simulink model "Lab2_Task_2"  (R2025b)
settings: Solver=FixedStepAuto  StartTime=0.0  StopTime=inf  RelTol=1e-3
model workspace (MAT data in the model file):
  SL_ROS_VariableLengthArrays_MaxSizes.CommonInfo.ArrayTruncateAction = 'EmitWarning'
  SL_ROS_VariableLengthArrays_MaxSizes.MsgTypeMap = containers.Map
  SL_ROS_VariableLengthArrays_MaxSizes.MsgTypeMap.serialization.keys = {'sensor_msgs/LaserScan'}
  SL_ROS_VariableLengthArrays_MaxSizes.MsgTypeMap.serialization.values{1}(1).PropertyName = 'intensities'
  SL_ROS_VariableLengthArrays_MaxSizes.MsgTypeMap.serialization.values{1}(1).DataType = 'single'
  SL_ROS_VariableLengthArrays_MaxSizes.MsgTypeMap.serialization.values{1}(1).MaxLength = 360
  SL_ROS_VariableLengthArrays_MaxSizes.MsgTypeMap.serialization.values{1}(2).PropertyName = 'ranges'
  SL_ROS_VariableLengthArrays_MaxSizes.MsgTypeMap.serialization.values{1}(2).DataType = 'single'
  SL_ROS_VariableLengthArrays_MaxSizes.MsgTypeMap.serialization.values{1}(2).MaxLength = 360
  SL_ROS_VariableLengthArrays_MaxSizes.MsgTypeMap.serialization.uniformity = 0
  SL_ROS_VariableLengthArrays_MaxSizes.MsgTypeMap.serialization.keyType = 'char'
  SL_ROS_VariableLengthArrays_MaxSizes.MsgTypeMap.serialization.valueType = 'any'
undefined symbols (not defined in the file or in its folder): header, twist
libraries: ros2lib x4
settings Model: Creator=scott  LastModifiedBy=abodynasser22
settings OptimizationCC: DefaultParameterBehavior=Inlined  EnhancedBackFolding=on  PassReuseOutputArgsAs=Individual arguments  ZeroExternalMemoryAtStartup=off  ZeroInternalMemoryAtStartup=off  MaxStackSize=64  OptimizeBlockOrder=speed  DifferentSizesBufferReuse=on  OptimizationCustomize=off  EfficientTunableParamExpr=on
settings DebuggingCC: ParameterTunabilityLossMsg=error
settings HardwareCC: ProdBitPerPointer=32.0  ProdBitPerSizeT=32.0  ProdBitPerPtrDiffT=32.0  ProdWordSize=32.0  ProdHWDeviceType=Intel->x86-32 (Windows32)  UseEmbeddedCoderFeatures=off
settings SFSimCC: MATLABDynamicMemAlloc=off
settings RTWCC: SystemTargetFile=ert.tlc  HardwareBoard=Robot Operating System 2 (ROS 2)  TLCOptions="-aInlineSetEventsForThisBaseRateFcn=TLC_FALSE -aSuppressMultiTaskScheduler=TLC_FALSE  -aRateBasedStepFcn=0"  TemplateMakefile=ert_default_tmf  Toolchain=Colcon Tools  TargetLang=C++  Description=Embedded Coder
settings CodeAppCC: ForceParamTrailComments=on  IgnoreCustomStorageClasses=off  OperatorAnnotations=on  SimulinkDataObjDesc=on  SFDataObjDesc=on  InsertBlockDesc=on
settings ERTTargetCC: ExtModeTransport=2.0  ExtModeStaticAlloc=on  ExtModeAutomaticAllocSize=off  ExtModeMexFile=ext_xcp  ExtModeIntrfLevel=Level2 - Open  RootIOFormat=Structure reference  CodeInterfacePackaging=C++ class  SupportNonInlinedSFcns=on

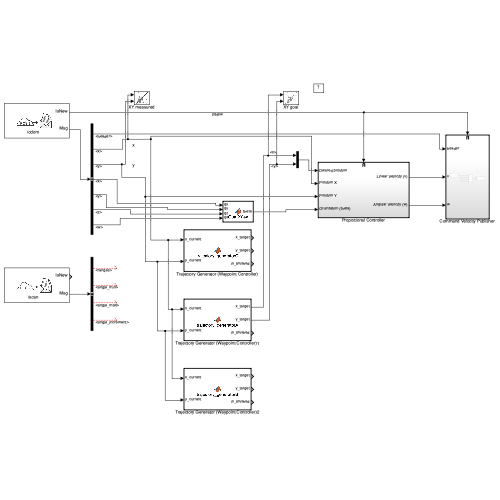
[thumbnail: Simulink's stored preview of the top-level diagram]
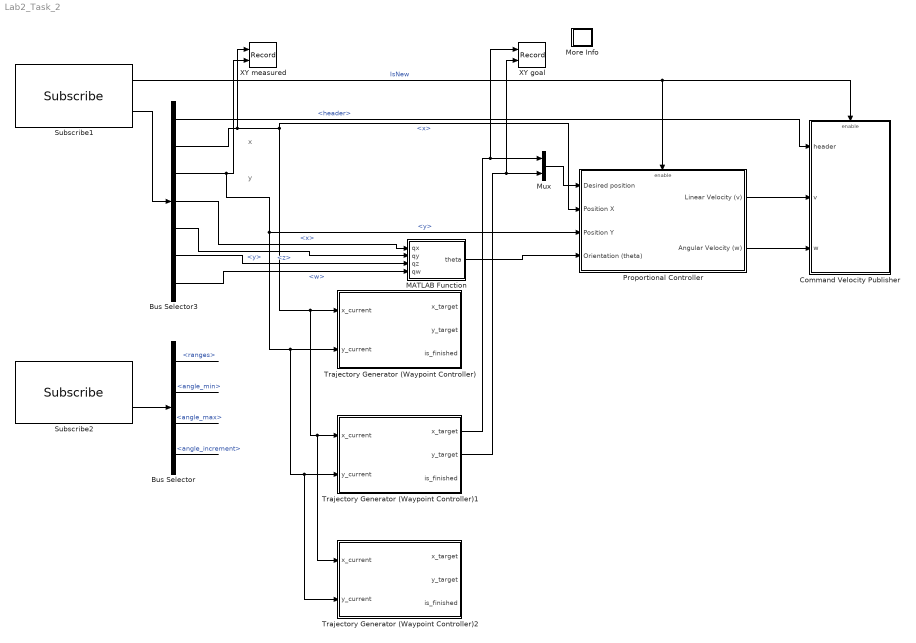
== system Lab2_Task_2 ==
  note: y
  note: x
  Bus Selector : BusSelector  OutputSignals=ranges,angle_min,angle_max,angle_increment
  Bus Selector3 : BusSelector  OutputSignals=header,pose.pose.position.x,pose.pose.position.y,pose.pose.orientation.x,pose.pose.orientation.y,pose.pose.orientation.z,pose.pose.orientation.w
  Command Velocity Publisher : Subsystem
  MATLAB Function : MATLAB Function  TreatAsAtomicUnit=on
  More Info : Subsystem
      settings: OpenFcn=showdemo(bdroot(gcb))
      mask Display: disp('?')
  Mux : Mux  Inputs=2
  Proportional Controller : Subsystem
  Subscribe1 : ros2lib/Subscribe  topicSource=Select from ROS network  topic=/odom  messageType=nav_msgs/Odometry  sampleTime=-1  QOSHistory=Keep last  QOSDepth=10  QOSReliability=Reliable  QOSDurability=Volatile  QOSDeadline=Inf  QOSLifespan=Inf  QOSLiveliness=Automatic  QOSLeaseDuration=Inf  QOSAvoidROSNamespaceConventions=off
  Subscribe2 : ros2lib/Subscribe  topicSource=Select from ROS network  topic=/scan  messageType=sensor_msgs/LaserScan  sampleTime=-1  QOSHistory=Keep last  QOSDepth=10  QOSReliability=Best effort  QOSDurability=Volatile  QOSDeadline=Inf  QOSLifespan=Inf  QOSLiveliness=Automatic  QOSLeaseDuration=Inf  QOSAvoidROSNamespaceConventions=off
  Trajectory Generator (Waypoint Controller) : MATLAB Function  TreatAsAtomicUnit=on
  Trajectory Generator (Waypoint Controller)1 : MATLAB Function  TreatAsAtomicUnit=on
  Trajectory Generator (Waypoint Controller)2 : MATLAB Function  TreatAsAtomicUnit=on
  XY goal : Record  NumPorts=2.0  FileSettingsInternal="{\"entries\":[{\"content\":{\"excelSettings\":{\"content\":{},\"type\":\"Streamout.ExcelSettings\"},\"parquetSettings\":{\"content\":{},\"type\":\"Streamout.ParquetSettings\"}},\"type\":\"Streamout.FileSettingStorage\",\"uuid\":\"\"}],\"packageUris\":[\"http:\\/\\/schema.mathworks.com\\/mf0\\/streamout_blocks\\/R2020a\"],\"version\":\"1.0\"}"  FrameSettings=[0, 0]  Layout=[1 1]  SignalsInternal="{\"entries\":[{\"content\":{\"signals\":[{\"content\":{\"blockPath\":[],\"dimensions\":[1],\"domain\":\"\",\"lineColor\":\"#a2142f\",\"plots\":[ 1 ],\"port\":1,\"signalID\":1,\"signalName\":\"<x>\"},\"type\":\"RecordBlkView.Signal\",\"uuid\":\"\"},{\"content\":{\"blockPath\":[],\"dimensions\":[1],\"domain\":\"\",\"lineColor\":\"#139fff\",\"plots\":[ 1 ],\"port\":2,\"signalID\":2,\"signalName\":\"<y>\"},\"type\":\"RecordBlkView.Signal\",\"uuid\":\"\"}]},\"type\":\"RecordBlkView.InputSignals\",\"uuid\":\"\"}],\"packageUris\":[\"http:\\/\\/schema.mathworks.com\\/mf0\\/streamout_blocks\\/R2020a\"],\"version\":\"1.0\"}"  VisualizationBindings="{\"xyplotplugin\":{\"info\":[{\"series\":[{\"bindingParametersList\":[{\"parameter\":\"X-Axis\",\"signalID\":1,\"signalName\":\"<x>;\"},{\"parameter\":\"Y-Axis\",\"signalID\":2,\"signalName\":\"<y>;\"}],\"seriesID\":0}],\"subplotID\":1}]}}"  CompatibilityTag=XY
  XY measured : Record  NumPorts=2.0  FileSettingsInternal="{\"entries\":[{\"content\":{\"excelSettings\":{\"content\":{},\"type\":\"Streamout.ExcelSettings\"},\"parquetSettings\":{\"content\":{},\"type\":\"Streamout.ParquetSettings\"}},\"type\":\"Streamout.FileSettingStorage\",\"uuid\":\"\"}],\"packageUris\":[\"http:\\/\\/schema.mathworks.com\\/mf0\\/streamout_blocks\\/R2020a\"],\"version\":\"1.0\"}"  FrameSettings=[0, 0]  Layout=[1 1]  SignalsInternal="{\"entries\":[{\"content\":{\"signals\":[{\"content\":{\"blockPath\":[],\"dimensions\":[1],\"domain\":\"\",\"lineColor\":\"#a2142f\",\"plots\":[ 1 ],\"port\":1,\"signalID\":1,\"signalName\":\"<x>\"},\"type\":\"RecordBlkView.Signal\",\"uuid\":\"\"},{\"content\":{\"blockPath\":[],\"dimensions\":[1],\"domain\":\"\",\"lineColor\":\"#139fff\",\"plots\":[ 1 ],\"port\":2,\"signalID\":2,\"signalName\":\"<y>\"},\"type\":\"RecordBlkView.Signal\",\"uuid\":\"\"}]},\"type\":\"RecordBlkView.InputSignals\",\"uuid\":\"\"}],\"packageUris\":[\"http:\\/\\/schema.mathworks.com\\/mf0\\/streamout_blocks\\/R2020a\"],\"version\":\"1.0\"}"  VisualizationBindings="{\"xyplotplugin\":{\"info\":[{\"series\":[{\"bindingParametersList\":[{\"parameter\":\"X-Axis\",\"signalID\":1,\"signalName\":\"<x>;\"},{\"parameter\":\"Y-Axis\",\"signalID\":2,\"signalName\":\"<y>;\"}],\"seriesID\":0}],\"subplotID\":1}]}}"  CompatibilityTag=XY
  wires:
  Subscribe1/2 -> Bus Selector3/1
  Subscribe1/1 -> Command Velocity Publisher/Enable, Proportional Controller/Enable  "IsNew"
  Proportional Controller/1(Linear Velocity (v)) -> Command Velocity Publisher/2(v)
  Proportional Controller/2(Angular Velocity (w)) -> Command Velocity Publisher/3(w)
  Bus Selector3/1 -> Command Velocity Publisher/1(header)  "<header>"
  Bus Selector3/2 -> XY measured/1, Trajectory Generator (Waypoint Controller)2/1(x_current), Trajectory Generator (Waypoint Controller)1/1(x_current), Trajectory Generator (Waypoint Controller)/1(x_current), Proportional Controller/2(Position X)  "<x>"
  Bus Selector3/3 -> XY measured/2, Trajectory Generator (Waypoint Controller)2/2(y_current), Trajectory Generator (Waypoint Controller)1/2(y_current), Trajectory Generator (Waypoint Controller)/2(y_current), Proportional Controller/3(Position Y)  "<y>"
  Bus Selector3/4 -> MATLAB Function/1(qx)  "<x>"
  Bus Selector3/5 -> MATLAB Function/2(qy)  "<y>"
  Bus Selector3/6 -> MATLAB Function/3(qz)  "<z>"
  Bus Selector3/7 -> MATLAB Function/4(qw)  "<w>"
  Subscribe2/2 -> Bus Selector/1
  Bus Selector/1 -> ?  "<ranges>"
  Bus Selector/2 -> ?  "<angle_min>"
  Bus Selector/3 -> ?  "<angle_max>"
  Bus Selector/4 -> ?  "<angle_increment>"
  MATLAB Function/1(theta) -> Proportional Controller/4(Orientation (theta))
  Mux/1 -> Proportional Controller/1(Desired position)
  Trajectory Generator (Waypoint Controller)1/1(x_target) -> XY goal/1, Mux/1
  Trajectory Generator (Waypoint Controller)1/2(y_target) -> XY goal/2, Mux/2

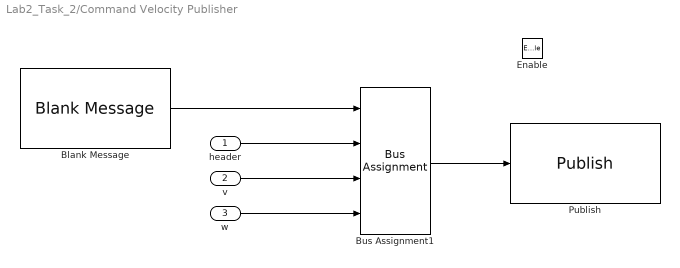
== system Lab2_Task_2/Command Velocity Publisher ==
  header : Inport
  v : Inport  Port=2
  w : Inport  Port=3
  Enable : EnablePort
  Blank Message : ros2lib/Blank Message  messageClass=Message  entityType=geometry_msgs/TwistStamped  messageType=geometry_msgs/TwistStamped  SampleTime=inf
  Bus Assignment1 : BusAssignment  DialogController=Simulink.DDGSource_BusAssignment  AssignedSignals=header,twist.linear.x,twist.angular.z
  Publish : ros2lib/Publish  topicSource=Select from ROS network  topic=/cmd_vel  messageType=geometry_msgs/TwistStamped  QOSHistory=Keep last  QOSDepth=10  QOSReliability=Reliable  QOSDurability=Volatile  QOSDeadline=Inf  QOSLifespan=Inf  QOSLiveliness=Automatic  QOSLeaseDuration=Inf  QOSAvoidROSNamespaceConventions=off
  wires:
  Bus Assignment1/1 -> Publish/1
  Blank Message/1 -> Bus Assignment1/1
  header/1 -> Bus Assignment1/2
  v/1 -> Bus Assignment1/3
  w/1 -> Bus Assignment1/4

== system Lab2_Task_2/More Info ==

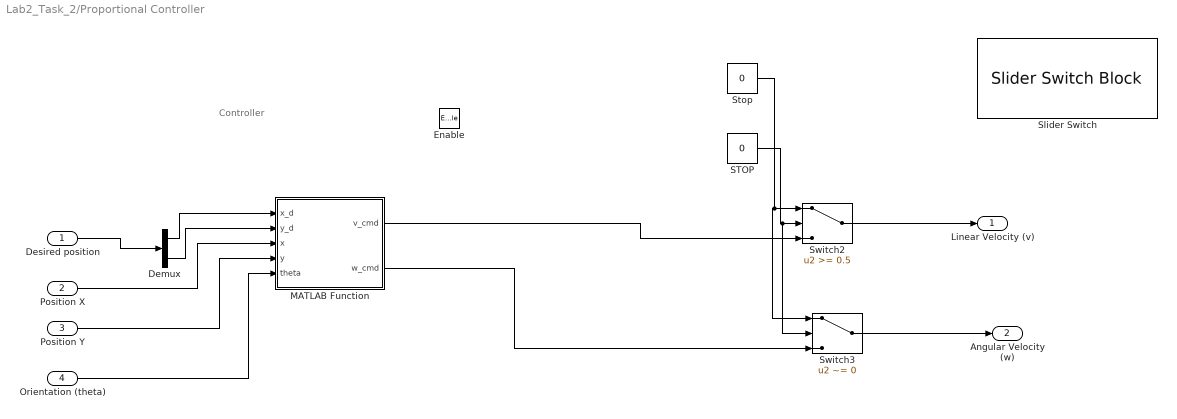
== system Lab2_Task_2/Proportional Controller ==
  note: Controller
  Desired position : Inport
  Position X : Inport  Port=2
  Position Y : Inport  Port=3
  Orientation (theta) : Inport  Port=4
  Enable : EnablePort
  Demux : Demux  Outputs=2
  MATLAB Function : MATLAB Function  TreatAsAtomicUnit=on
  "STOP " : Constant  Value=0
  Slider Switch : SliderSwitchBlock
  Stop : Constant  Value=0
  Switch2 : Switch  Threshold=0.5  SaturateOnIntegerOverflow=off  InputSameDT=off
  Switch3 : Switch  Criteria=u2 ~= 0  Threshold=0.5  SaturateOnIntegerOverflow=off  InputSameDT=off
  Linear Velocity (v) : Outport  VectorParamsAs1DForOutWhenUnconnected=off
  Angular Velocity (w) : Outport  Port=2  VectorParamsAs1DForOutWhenUnconnected=off
  wires:
  Stop/1 -> Switch3/1, Switch2/1
  "STOP "/1 -> Switch3/2, Switch2/2
  Switch2/1 -> Linear Velocity (v)/1
  Switch3/1 -> Angular Velocity (w)/1
  Desired position/1 -> Demux/1
  Demux/1 -> MATLAB Function/1(x_d)
  Demux/2 -> MATLAB Function/2(y_d)
  Position Y/1 -> MATLAB Function/4(y)
  Position X/1 -> MATLAB Function/3(x)
  MATLAB Function/1(v_cmd) -> Switch2/3
  Orientation (theta)/1 -> MATLAB Function/5(theta)
  MATLAB Function/2(w_cmd) -> Switch3/3

== matlab function Lab2_Task_2/MATLAB Function ==
  data: qx input; theta output; qy input; qz input; qw input
function theta = Quat2Yaw(qx, qy, qz, qw)
%#codegen
% Inputs are quaternion components from /odom:
% orientation.x = qx, .y = qy, .z = qz, .w = qw

% Build 1x4 quaternion row in the order [w x y z]
q = [qw, qx, qy, qz];

% Convert to Euler angles [yaw pitch roll] (ZYX convention)
eul = quat2eul(q, 'ZYX');

% Use yaw (rotation about Z-axis)
theta = eul(1);
end

== matlab function Lab2_Task_2/Proportional Controller/MATLAB Function ==
  data: x_d input; v_cmd output; y_d input; x input; y input; theta input; w_cmd output
function [v_cmd, w_cmd] = pose_controller(x_d, y_d, x, y, theta)
%#codegen
% Enkel P-regulator för differentialdriven robot

% --- parametrar (tune vid behov) ---
Kv = 0.6;      % linjär hastighetsförstärkning
Kw = 1.5;      % vinkelhastighetsförstärkning
d_stop = 0.05; % stopp-radie [m]

% --- fel i position ---
dx = x_d - x;
dy = y_d - y;

% Avstånd till mål
d = sqrt(dx^2 + dy^2);

% Vinkel mot mål i världssystemet
theta_goal = atan2(dy, dx);

% Vinkelfel (wrap till [-pi, pi])
alpha = theta_goal - theta;      
alpha = atan2(sin(alpha), cos(alpha));

% --- P-lagar ---
v_cmd = Kv * d;       %Velocity (Linjär hastigher)
w_cmd = Kw * alpha;   %Angular Velocity (Vinkel hastighet)

% --- Stanna när vi är nära målet ---
if d < d_stop
    v_cmd = 0;
    w_cmd = 0;
end
end

== matlab function Lab2_Task_2/Trajectory Generator (Waypoint Controller) ==
  data: x_current input; y_current input; x_target output; y_target output; is_finished output
function [x_target, y_target, is_finished] = trajectory_generatorC(x_current, y_current)
%#codegen
% Följer en sinusformad bana definierad av waypoint_list.
% Använder segment-projektion + look-ahead för mjuk följning.

    % ----------------------------------------------------------
    % PERSISTENT VARIABLES (sparas mellan tidssteg)
    % ----------------------------------------------------------
    persistent waypoint_list
    persistent segment_index
    persistent waypoint_reach_tolerance
    persistent lookahead_distance
    persistent completed

    % ----------------------------------------------------------
    % INITIALISERING (körs bara första gången)
    % ----------------------------------------------------------
    if isempty(waypoint_list)
        % ----- Generera sinusformade waypoints (samma som din grundidé) -----
        x_offset    = 0.0;
        y_offset    = 0.0;
        path_length = 2.0;   % m
        A           = 0.3;   % amplitud
        num_waves   = 1.0;   % antal fulla sinusvågor

        num_points = 20;                                % antal diskreta punkter
        s_values   = linspace(0, path_length, num_points)';  % kolumn

        k = 2 * pi * num_waves / path_length;

        x_points = x_offset + s_values;
        y_points = y_offset + A * sin(k * s_values);

        waypoint_list = [x_points, y_points];

        % ----- Parametrar för följning -----
        segment_index = 1;
        waypoint_reach_tolerance = 0.05;   % m
        lookahead_distance       = 0.15;   % m (finjustera vid behov)
        completed = false;
    end

    % ----------------------------------------------------------
    % Om banan är klar: håll sista punkt
    % ----------------------------------------------------------
    if completed
        x_target    = waypoint_list(end,1);
        y_target    = waypoint_list(end,2);
        is_finished = true;
        return;
    end

    % ----------------------------------------------------------
    % Antal waypoints och säkerhetskontroll
    % ----------------------------------------------------------
    N = size(waypoint_list, 1);

    if segment_index >= N
        px = waypoint_list(N,1);
        py = waypoint_list(N,2);
        x_target = px;
        y_target = py;

        dist_last = hypot(x_current - px, y_current - py);
        if dist_last < waypoint_reach_tolerance
            completed   = true;
            is_finished = true;
        else
            is_finished = false;
        end
        return;
    end

    % ----------------------------------------------------------
    % 1) Aktuellt segment P1 -> P2
    % ----------------------------------------------------------
    p1x = waypoint_list(segment_index,   1);
    p1y = waypoint_list(segment_index,   2);
    p2x = waypoint_list(segment_index+1, 1);
    p2y = waypoint_list(segment_index+1, 2);

    sx = p2x - p1x;
    sy = p2y - p1y;
    L  = hypot(sx, sy);

    if L < 1e-6
        % Degenererat segment, hoppa vidare
        segment_index = segment_index + 1;
        x_target = p2x;
        y_target = p2y;
        is_finished = false;
        return;
    end

    % ----------------------------------------------------------
    % 2) Projektion av robotens position på segmentet
    % ----------------------------------------------------------
    rx = x_current - p1x;
    ry = y_current - p1y;

    t = (rx * sx + ry * sy) / (L * L);
    if t < 0
        t = 0;
    elseif t > 1
        t = 1;
    end

    xc = p1x + t * sx;
    yc = p1y + t * sy;

    % ----------------------------------------------------------
    % 3) Look-ahead längs segmentet
    % ----------------------------------------------------------
    dt       = lookahead_distance / L;
    t_target = t + dt;
    if t_target > 1
        t_target = 1;
    end

    x_target = p1x + t_target * sx;
    y_target = p1y + t_target * sy;

    % ----------------------------------------------------------
    % 4) Byt segment när vi är nära nästa punkt
    % ----------------------------------------------------------
    dist_to_p2 = hypot(x_current - p2x, y_current - p2y);
    corner_switch_dist = 0.10;   % m, justera vid behov

    if (dist_to_p2 < corner_switch_dist) && (segment_index < N-1)
        segment_index = segment_index + 1;
    end

    % ----------------------------------------------------------
    % 5) Kolla om vi är klara med sista waypoint
    % ----------------------------------------------------------
    if segment_index == N-1
        last_x = waypoint_list(N,1);
        last_y = waypoint_list(N,2);
        dist_last = hypot(x_current - last_x, y_current - last_y);

        if dist_last < waypoint_reach_tolerance
            completed   = true;
            is_finished = true;
            x_target    = last_x;
            y_target    = last_y;
            return;
        end
    end

    is_finished = false;
end

== matlab function Lab2_Task_2/Trajectory Generator (Waypoint Controller)1 ==
  data: x_current input; y_current input; x_target output; y_target output; is_finished output
function [x_target, y_target, is_finished] = trajectory_generatorA(x_current, y_current)
%#codegen
% Genererar en referenspunkt som glider längs en brytlinje av waypoints.
% I stället för att alltid sikta direkt på en diskret waypoint används
% projektion på aktuellt linjesegment + look-ahead för att göra svängarna
% mjukare och minska överkompensation.

    % ----------------------------------------------------------
    % PERSISTENT VARIABLES (sparas mellan tidssteg)
    % ----------------------------------------------------------
    persistent waypoint_list           % [N x 2] lista av waypoints
    persistent segment_index           % index på aktuellt segment (i -> i+1)
    persistent waypoint_reach_tol      % tolerans för att anse banan klar
    persistent lookahead_distance      % hur långt fram på segmentet vi siktar
    persistent completed               % flagga när hela banan är klar

    % ----------------------------------------------------------
    % INITIALISERING (körs bara första gången)
    % ----------------------------------------------------------
    if isempty(waypoint_list)
        % Definiera waypoints (samma som tidigare, kvadrat)
        waypoint_list = [ 0.0  0.0;   % start
                          0.5  0.0;
                          0.5  0.5;
                          0.0  0.5;
                          0.0  0.0];  % tillbaka till start
        
        % Vi startar på segment 1: from waypoint 1 -> 2
        segment_index = 1;
        
        % Ungefär när roboten är "tillräckligt nära" sista punkten
        waypoint_reach_tol = 0.05;   % m
        
        % Look-ahead längs segmentet (kan finjusteras)
        lookahead_distance = 0.15;   % m
        
        completed = false;
    end

    % ----------------------------------------------------------
    % Om banan är klar: håll sista punkt
    % ----------------------------------------------------------
    if completed
        x_target   = waypoint_list(end, 1);
        y_target   = waypoint_list(end, 2);
        is_finished = true;
        return;
    end

    % Antal waypoints
    N = size(waypoint_list, 1);

    % Säkerhet: om segment_index är vid slutet → bara sikta på sista punkt
    if segment_index >= N
        px = waypoint_list(N,1);
        py = waypoint_list(N,2);
        x_target = px;
        y_target = py;
        
        dist_last = hypot(x_current - px, y_current - py);
        if dist_last < waypoint_reach_tol
            completed   = true;
            is_finished = true;
        else
            is_finished = false;
        end
        return;
    end

    % ----------------------------------------------------------
    % 1) Hämta aktuellt segment: P1 -> P2
    % ----------------------------------------------------------
    p1x = waypoint_list(segment_index,   1);
    p1y = waypoint_list(segment_index,   2);
    p2x = waypoint_list(segment_index+1, 1);
    p2y = waypoint_list(segment_index+1, 2);

    sx = p2x - p1x;
    sy = p2y - p1y;
    L  = hypot(sx, sy);

    % Om segmentet i princip är noll långt: hoppa vidare
    if L < 1e-6
        segment_index = segment_index + 1;
        % Kör funktionen igen nästa tidssteg, här gör vi enkel fallback:
        x_target   = p2x;
        y_target   = p2y;
        is_finished = false;
        return;
    end

    % ----------------------------------------------------------
    % 2) Projicera robotens position på linjesegmentet
    % ----------------------------------------------------------
    % Position relativt P1
    rx = x_current - p1x;
    ry = y_current - p1y;

    % Parameter t längs segmentet (linje), 0 = P1, 1 = P2
    t = (rx * sx + ry * sy) / (L * L);

    % Klampa till segmentet [0, 1]
    if t < 0
        t = 0;
    elseif t > 1
        t = 1;
    end

    % Närmaste punkt på segmentet
    xc = p1x + t * sx;
    yc = p1y + t * sy;

    % ----------------------------------------------------------
    % 3) Look-ahead: siktpunkten ligger en bit längre fram än projicerad punkt
    % ----------------------------------------------------------
    % Hur stor del av segmentet motsvarar lookahead_distance?
    dt = lookahead_distance / L;
    t_target = t + dt;
    if t_target > 1
        t_target = 1;
    end

    x_target = p1x + t_target * sx;
    y_target = p1y + t_target * sy;

    % ----------------------------------------------------------
    % 4) Avancera till nästa segment när vi passerat hörnet
    % ----------------------------------------------------------
    % Om vi är nära nästa waypoint (P2) → byt till nästa segment
    dist_to_p2 = hypot(x_current - p2x, y_current - p2y);

    % Detta “corner_switch_dist” kan göras större än waypoint_reach_tol
    % om du vill börja svänga ännu tidigare.
    corner_switch_dist = 0.10;   % m, kan justeras

    if (dist_to_p2 < corner_switch_dist) && (segment_index < N-1)
        segment_index = segment_index + 1;
    end

    % ----------------------------------------------------------
    % 5) Kontroll om vi är klara med sista punkt
    % ----------------------------------------------------------
    if segment_index == N-1
        % Sista segmentet; om roboten är nära sista waypoint → klar
        last_x = waypoint_list(N,1);
        last_y = waypoint_list(N,2);
        dist_last = hypot(x_current - last_x, y_current - last_y);

        if dist_last < waypoint_reach_tol
            completed    = true;
            is_finished  = true;
            % sätt referensen exakt till sista punkten
            x_target = last_x;
            y_target = last_y;
            return;
        end
    end

    is_finished = false;
end

== matlab function Lab2_Task_2/Trajectory Generator (Waypoint Controller)2 ==
  data: x_current input; y_current input; x_target output; y_target output; is_finished output
function [x_target, y_target, is_finished] = trajectory_generatorB(x_current, y_current)
%#codegen
% Följer en polygonbana definierad av waypoint_list med
% segment-projektion + look-ahead för mjukare svängar.

    % ----------------------------------------------------------
    % PERSISTENT VARIABLES (sparas mellan tidssteg)
    % ----------------------------------------------------------
    persistent waypoint_list
    persistent segment_index
    persistent waypoint_reach_tolerance
    persistent lookahead_distance
    persistent completed

    % ----------------------------------------------------------
    % INITIALISERING (körs bara första gången)
    % ----------------------------------------------------------
    if isempty(waypoint_list)
        % Waypoints för 2b (rätta till som Nx2-matris)
        waypoint_list = [  0.5    0.70;   % 2b)
                           0.5    1.00;
                           0.0    1.00;
                           0.0    0.0;
                           0.5    0.0;
                           0.5    0.5;
                          -0.25   0.5 ];

        segment_index = 1;          % starta på segment 1 -> 2
        waypoint_reach_tolerance = 0.05;   % m, när vi är "klara" med sista punkt
        lookahead_distance       = 0.15;   % m, justera vid behov
        completed = false;
    end

    % ----------------------------------------------------------
    % Om banan är klar: håll sista punkt
    % ----------------------------------------------------------
    if completed
        x_target    = waypoint_list(end,1);
        y_target    = waypoint_list(end,2);
        is_finished = true;
        return;
    end

    % ----------------------------------------------------------
    % Antal waypoints och säkerhetskontroll
    % ----------------------------------------------------------
    N = size(waypoint_list, 1);

    if segment_index >= N
        % Vi har passerat sista segmentet, bara sikta på sista punkt
        px = waypoint_list(N,1);
        py = waypoint_list(N,2);
        x_target = px;
        y_target = py;

        dist_last = hypot(x_current - px, y_current - py);
        if dist_last < waypoint_reach_tolerance
            completed   = true;
            is_finished = true;
        else
            is_finished = false;
        end
        return;
    end

    % ----------------------------------------------------------
    % 1) Aktuellt segment P1 -> P2
    % ----------------------------------------------------------
    p1x = waypoint_list(segment_index,   1);
    p1y = waypoint_list(segment_index,   2);
    p2x = waypoint_list(segment_index+1, 1);
    p2y = waypoint_list(segment_index+1, 2);

    sx = p2x - p1x;
    sy = p2y - p1y;
    L  = hypot(sx, sy);

    if L < 1e-6
        % Degenererat segment, hoppa vidare
        segment_index = segment_index + 1;
        x_target = p2x;
        y_target = p2y;
        is_finished = false;
        return;
    end

    % ----------------------------------------------------------
    % 2) Projektion av robotens position på segmentet
    % ----------------------------------------------------------
    rx = x_current - p1x;
    ry = y_current - p1y;

    t = (rx * sx + ry * sy) / (L * L);   % linjeparameter
    if t < 0
        t = 0;
    elseif t > 1
        t = 1;
    end

    xc = p1x + t * sx;
    yc = p1y + t * sy;

    % ----------------------------------------------------------
    % 3) Look-ahead längs segmentet
    % ----------------------------------------------------------
    dt       = lookahead_distance / L;
    t_target = t + dt;
    if t_target > 1
        t_target = 1;
    end

    x_target = p1x + t_target * sx;
    y_target = p1y + t_target * sy;

    % ----------------------------------------------------------
    % 4) Byt segment när vi är nära nästa hörn (P2)
    % ----------------------------------------------------------
    dist_to_p2 = hypot(x_current - p2x, y_current - p2y);
    corner_switch_dist = 0.10;   % m, justera vid behov

    if (dist_to_p2 < corner_switch_dist) && (segment_index < N-1)
        segment_index = segment_index + 1;
    end

    % ----------------------------------------------------------
    % 5) Kolla om vi är klara med sista waypoint
    % ----------------------------------------------------------
    if segment_index == N-1
        last_x = waypoint_list(N,1);
        last_y = waypoint_list(N,2);
        dist_last = hypot(x_current - last_x, y_current - last_y);

        if dist_last < waypoint_reach_tolerance
            completed   = true;
            is_finished = true;
            x_target    = last_x;
            y_target    = last_y;
            return;
        end
    end

    is_finished = false;
end
